simulink model "quarter_car_msd_2x"  (R2026b)
settings: Solver=ode23t  StopTime=25  MaxStep=5e-3  AbsTol=1e-3  EnableMultiTasking=on
PreLoadFcn:
  | quarter_car_msd_2x_param
  | load testrig_AirOilPiston_roughroad
values from neighbouring files (symbols this model uses):
  c_s = c_s_stiff    [offroad_ex01_msd.m]    (also in quarter_car_msd_2x_param.m = 2*zeta*sqrt(k_s*m_s))
  g = 9.81    [quarter_car_msd_2x_param.m]
  k_t = k_eq-k_s    (= 397587.143693)    [quarter_car_msd_2x_param.m]
  m_s = m_tot - m_us    (= 419.625)    [quarter_car_msd_2x_param.m]
  m_tot = 1865/4    (= 466.25)    [quarter_car_msd_2x_param.m]
  m_us = 0.1*m_tot    (= 46.625)    [quarter_car_msd_2x_param.m]
libraries: fl_lib x23, nesl_utility x5, testrig_AirOilPiston_lib x1
settings Model: Creator=smiller  LastModifiedBy=smiller
settings SolverCC: AutoScaleAbsTol=off
settings DataIOCC: LimitDataPoints=on  MaxDataPoints=10000  ReturnWorkspaceOutputs=off  SignalLoggingName=logsout_quarter_car_msd_2x
settings OptimizationCC: LifeSpan=inf
settings DebuggingCC: AllowSymbolicDim=off  ArithmeticOperatorsInVariantConditions=warning  SFExecutionAtInitializationDiag=none  SFNoUnconditionalDefaultTransitionDiag=warning  SFUnexpectedBacktrackingDiag=warning
settings SFSimCC: CustomCodeUndefinedFunction=UseInterfaceOnly  SimUseLocalCustomCode=off
settings RTWCC: DLArmComputeVersion=19.05  RTWUseLocalCustomCode=off
settings CodeAppCC: StateflowObjectComments=on
settings GRTTargetCC: TargetLangStandard=C89/C90 (ANSI)
settings ConfigComp: CovExternalEMLEnable=off  CovSFcnEnable=off  CovSaveCumulativeToWorkspaceVar=on  CovSaveSingleToWorkspaceVar=on
settings SimscapeCC: SimscapeLogName=simlog_quarter_car_msd_2x  SimscapeLogSimulationStatistics=on  SimscapeLogType=all  SimscapeUseEnergyAccounting=off

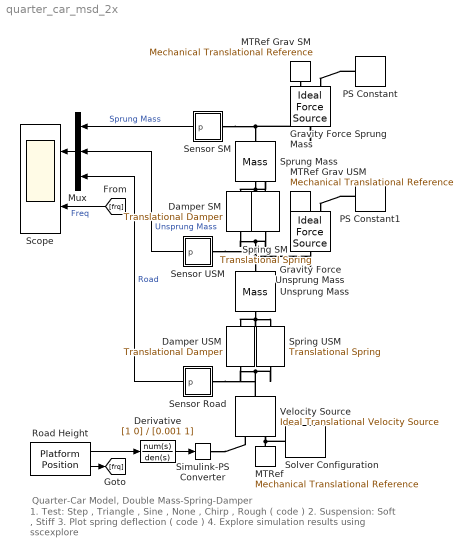
== system quarter_car_msd_2x ==
  note: Quarter-Car Model, Double Mass-Spring-Damper
  note: 1. Test: Step , Triangle , Sine , None , Chirp , Rough ( code )
      | 2. Suspension: Soft , Stiff
      | 3. Plot spring deflection ( code )
      | 4. Explore simulation results using sscexplore
  Damper SM : fl_lib/Mechanical/Translational Elements/Translational Damper  D=c_s N*s/m  v_specify=off  v_priority=None  v=0 m/s  v_nominal_specify=off  v_nominal_value=1  v_nominal_unit=m/s  f_specify=off  f_priority=None  f=0 N  f_nominal_specify=off  f_nominal_value=1  f_nominal_unit=N
  Damper USM : fl_lib/Mechanical/Translational Elements/Translational Damper  D=k_t/10 N*s/m  v_specify=off  v_priority=None  v=0 m/s  v_nominal_specify=off  v_nominal_value=1  v_nominal_unit=m/s  f_specify=off  f_priority=None  f=0 N  f_nominal_specify=off  f_nominal_value=1  f_nominal_unit=N
  Derivative : TransferFcn  Numerator=[1 0]  Denominator=[0.001 1]
  Gravity Force Sprung Mass : fl_lib/Mechanical/Mechanical Sources/Ideal Force Source
  Gravity Force Unsprung Mass : fl_lib/Mechanical/Mechanical Sources/Ideal Force Source
  MTRef : fl_lib/Mechanical/Translational Elements/Mechanical Translational Reference
  MTRef Grav SM : fl_lib/Mechanical/Translational Elements/Mechanical Translational Reference
  MTRef Grav USM : fl_lib/Mechanical/Translational Elements/Mechanical Translational Reference
  Mux : Mux  Inputs=3
  PS Constant : fl_lib/Physical Signals/Sources/PS Constant  constant=-m_s*g N
  PS Constant1 : fl_lib/Physical Signals/Sources/PS Constant  constant=-m_us*g N
  Road Height : testrig_AirOilPiston_lib/Inputs/Platform Position  popup_signalType=Step  tPer=4  chirpFreqStart=0.5  chirpFreqFinish=5  chirpTimeStart=5  chirpTimeFinish=20  pAmp=0.05  nCyc=50  nCycSet=1  spdkmh=10  roughTimeStart=5
      settings: AttributesFormatString=%<popup_signalType>
  "Scope " : Scope  NumInputPorts=2
      settings: Title=Vertical Positions  ActiveDisplayYMinimum=-0.1266  ActiveDisplayYMaximum=0.2266
  Sensor Road : Subsystem
  Sensor SM : Subsystem
  Sensor USM : Subsystem
  Simulink-PS Converter : nesl_utility/Simulink-PS Converter  PhysicalDomain=network_engine_domain  SubClassName=ps_input  LeftPortType=input  RightPortType=output  PseudoPeriodic=off  Frequencies=[]  NoiseDistribution=none  NoiseParameters=[]  Unit=1  AffineConversion=off  FilteringAndDerivatives=provide  SimscapeFilterOrder=1  InputFilterTimeConstant=0.001  UdotUserProvided=0
  Solver Configuration : nesl_utility/Solver Configuration  PhysicalDomain=network_engine_domain  SubClassName=solver  LeftPortType=input  RightPortType=generic  Tones=[]  Harmonics=[]  SimulateNoise=off  Profile=off  UseLocalSampling=off  EnableSwitchedLinearOptims=on  FrequencyDomain=off  UseCCode=off  RelTol=0.001  AbsTol=1e-06  MinStep=1e-09  ToWorkspace=off  RevertToSquareIcSolve=off  NumHomotopyIterations=100  PhasorMode=off  PhasorModeNumHarmonics=1  ConsistencySolver=NEWTON_FTOL  CanonicalOrdering=UNORDERED  OptimizeIntermediates=UNOPTIMIZED  MulticoreSolverChoice=BACKWARD_EULER  IndexReductionMethod=DerivativeReplacement  DoDC=off  ResidualTolerance=1e-09  ConsistencyTolSource=GLOBAL  ConsistencyAbsTol=0.001  ConsistencyRelTol=0.001  ConsistencyTolFactor=0.001  UseLocalSolver=off  LocalSolverChoice=NE_BACKWARD_EULER_ADVANCER  ResolveIndetEquations=on  FunctionEvalNumThread=1  LocalSolverSampleTime=0.001  DoFixedCost=off  MaxNonlinIter=3  MaxModeIter=2  ComputeImpulses=off  ImpulseIterations=2  LinearAlgebra=Sparse  LinearAlgebraNumThread=0  EquationFormulation=NE_TIME_EF  DelaysMemoryBudget=1024  AutomaticFiltering=on  FilteringTimeConstant=0.001  PartitionStorageMethod=AS_NEEDED  PartitionMemoryBudget=1024  PartitionMethod=FAST  MultibodyUseLocalSolver=off  MultibodyLocalSolverChoice=ODE1  MultibodyLocalSolverSampleTime=0.001
  Spring SM : fl_lib/Mechanical/Translational Elements/Translational Spring  spr_rate=k_s N/m  v_specify=off  v_priority=None  v=0 m/s  v_nominal_specify=off  v_nominal_value=1  v_nominal_unit=m/s  f_specify=on  f_priority=High  f=-m_s*g N  f_nominal_specify=off  f_nominal_value=1  f_nominal_unit=N  x_specify=on  x_priority=None  x=0 m  x_nominal_specify=off  x_nominal_value=1  x_nominal_unit=m
  Spring USM : fl_lib/Mechanical/Translational Elements/Translational Spring  spr_rate=k_t N/m  v_specify=off  v_priority=None  v=0 m/s  v_nominal_specify=off  v_nominal_value=1  v_nominal_unit=m/s  f_specify=on  f_priority=High  f=-m_tot*g N  f_nominal_specify=off  f_nominal_value=1  f_nominal_unit=N  x_specify=on  x_priority=None  x=0 m  x_nominal_specify=off  x_nominal_value=1  x_nominal_unit=m
  Sprung Mass : fl_lib/Mechanical/Translational Elements/Mass  mass=m_s kg  num_ports=foundation.enum.numPorts2.two  v_specify=off  v_priority=High  v=0 m/s  v_nominal_specify=off  v_nominal_value=1  v_nominal_unit=m/s  f_specify=off  f_priority=None  f=0 N  f_nominal_specify=off  f_nominal_value=1  f_nominal_unit=N
  Unsprung Mass : fl_lib/Mechanical/Translational Elements/Mass  mass=m_us kg  num_ports=foundation.enum.numPorts2.two  v_specify=off  v_priority=High  v=0 m/s  v_nominal_specify=off  v_nominal_value=1  v_nominal_unit=m/s  f_specify=off  f_priority=None  f=0 N  f_nominal_specify=off  f_nominal_value=1  f_nominal_unit=N
  Velocity Source : fl_lib/Mechanical/Mechanical Sources/Ideal Translational Velocity Source
  wires:
  Sensor USM/1(p) -> Mux/2  "Unsprung Mass"
  Derivative/1 -> Simulink-PS Converter/1
  Road Height/1 -> Derivative/1
  Sensor SM/1(p) -> Mux/1  "Sprung Mass"
  Sensor Road/1(p) -> Mux/3  "Road"
  Road Height/2 -> [frq]
  Mux/1 -> "Scope "/1
  [frq] -> "Scope "/2  "Freq"
  connections:
  Spring USM/RConn1 -- Sensor Road/LConn1 -- Velocity Source/LConn1 -- Damper USM/RConn1
  Unsprung Mass/RConn1 -- Spring USM/LConn1 -- Damper USM/LConn1
  MTRef/LConn1 -- Solver Configuration/RConn1 -- Velocity Source/RConn2
  Damper SM/RConn1 -- Sensor USM/LConn1 -- Gravity Force Unsprung Mass/LConn1 -- Unsprung Mass/LConn1 -- Spring SM/RConn1
  Spring SM/LConn1 -- Damper SM/LConn1 -- Sprung Mass/RConn1
  Simulink-PS Converter/RConn1 -- Velocity Source/RConn1
  PS Constant/RConn1 -- Gravity Force Sprung Mass/RConn1
  MTRef Grav SM/LConn1 -- Gravity Force Sprung Mass/RConn2
  PS Constant1/RConn1 -- Gravity Force Unsprung Mass/RConn1
  MTRef Grav USM/LConn1 -- Gravity Force Unsprung Mass/RConn2
  Gravity Force Sprung Mass/LConn1 -- Sprung Mass/LConn1 -- Sensor SM/LConn1

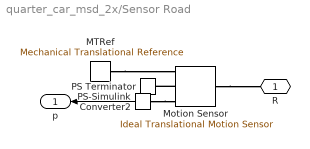
== system quarter_car_msd_2x/Sensor Road ==
  MTRef : fl_lib/Mechanical/Translational Elements/Mechanical Translational Reference
  Motion Sensor : fl_lib/Mechanical/Mechanical Sensors/Ideal Translational Motion Sensor  reference=foundation.enum.MeasurementReference.difference  acceleration_port=false  velocity_port=true  position_port=true  offset=0 m
  PS Terminator : fl_lib/Physical Signals/Sinks/PS Terminator
  PS-Simulink Converter2 : nesl_utility/PS-Simulink Converter  PhysicalDomain=network_engine_domain  SubClassName=ps_output  LeftPortType=input  RightPortType=output  PseudoPeriodic=off  Frequencies=[]  VectorFormat=inherit  Unit=inherit  AffineConversion=off
  R : PMIOPort  Side=Left
  p : Outport
  wires:
  PS-Simulink Converter2/1 -> p/1
  connections:
  PS-Simulink Converter2/LConn1 -- Motion Sensor/RConn3
  Motion Sensor/RConn2 -- PS Terminator/LConn1
  MTRef/LConn1 -- Motion Sensor/RConn1
  Motion Sensor/LConn1 -- R/RConn1

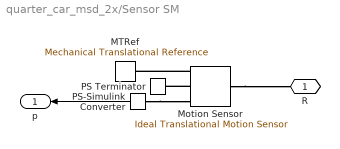
== system quarter_car_msd_2x/Sensor SM ==
  MTRef : fl_lib/Mechanical/Translational Elements/Mechanical Translational Reference
  Motion Sensor : fl_lib/Mechanical/Mechanical Sensors/Ideal Translational Motion Sensor  reference=foundation.enum.MeasurementReference.difference  acceleration_port=false  velocity_port=true  position_port=true  offset=0 m
  PS Terminator : fl_lib/Physical Signals/Sinks/PS Terminator
  PS-Simulink Converter : nesl_utility/PS-Simulink Converter  PhysicalDomain=network_engine_domain  SubClassName=ps_output  LeftPortType=input  RightPortType=output  PseudoPeriodic=off  Frequencies=[]  VectorFormat=inherit  Unit=inherit  AffineConversion=off
  R : PMIOPort  Side=Left
  p : Outport
  wires:
  PS-Simulink Converter/1 -> p/1
  connections:
  Motion Sensor/RConn1 -- MTRef/LConn1
  PS-Simulink Converter/LConn1 -- Motion Sensor/RConn3
  Motion Sensor/LConn1 -- R/RConn1
  Motion Sensor/RConn2 -- PS Terminator/LConn1

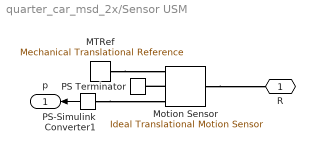
== system quarter_car_msd_2x/Sensor USM ==
  MTRef : fl_lib/Mechanical/Translational Elements/Mechanical Translational Reference
  Motion Sensor : fl_lib/Mechanical/Mechanical Sensors/Ideal Translational Motion Sensor  reference=foundation.enum.MeasurementReference.difference  acceleration_port=false  velocity_port=true  position_port=true  offset=0 m
  PS Terminator : fl_lib/Physical Signals/Sinks/PS Terminator
  PS-Simulink Converter1 : nesl_utility/PS-Simulink Converter  PhysicalDomain=network_engine_domain  SubClassName=ps_output  LeftPortType=input  RightPortType=output  PseudoPeriodic=off  Frequencies=[]  VectorFormat=inherit  Unit=inherit  AffineConversion=off
  R : PMIOPort  Side=Left
  p : Outport
  wires:
  PS-Simulink Converter1/1 -> p/1
  connections:
  PS-Simulink Converter1/LConn1 -- Motion Sensor/RConn3
  Motion Sensor/RConn2 -- PS Terminator/LConn1
  MTRef/LConn1 -- Motion Sensor/RConn1
  Motion Sensor/LConn1 -- R/RConn1
